simulink model "CLVF"  (R2020a)
settings: Solver=FixedStepAuto  StartTime=0.0  StopTime=tsim  FixedStep=baseRate  RelTol=1e-3  EnableMultiTasking=on
values from neighbouring files (symbols this model uses):
  a = sqrt(sum(aTimesOVec.^2))    [Run_Initializer.m]    (also in a_max_CLVF2D.m = params(4))
  a_max = 0.4/BLACKMass    [Run_Initializer.m]
  a_prime = newParams(2)    [Run_Initializer.m]    (also in a_max_LVF.m = params(2))
  acceptableRadius = 0.05    [Run_Initializer.m]
  b = newParams(3)    [Run_Initializer.m]    (also in a_max_CLVF2D.m = params(3))
  baseRate = 0.05    [Run_Initializer.m]
  BLACKMass = model_param(3)    [Run_Initializer.m]
  d = [0.16;0.542;0]    [Run_Initializer.m]    (also in a_max_LVF.m = [rotStuff(3);rotStuff(4);rotStuff(5)])
  drop_states_BLACK = rC_I0    [Run_Initializer.m]
  drop_states_BLUE = [ xLength/2+0.9; yLength/2+0.5; 0]    [Run_Initializer.m]
  drop_states_RED = rT_I0    [Run_Initializer.m]
  F_thrusters_BLACK = 0.25.*ones(8,1)    [Run_Initializer.m]
  F_thrusters_BLUE = 0.25.*ones(8,1)    [Run_Initializer.m]
  F_thrusters_RED = 0.25.*ones(8,1)    [Run_Initializer.m]
  home_states_BLACK = [ xLength/2+0.4; yLength/2; 0]    [Run_Initializer.m]
  home_states_BLUE = [ xLength/2-0.9; yLength/2+0.5; 0]    [Run_Initializer.m]
  home_states_RED = [ xLength/2-0.4; yLength/2; 0]    [Run_Initializer.m]
  init_states_BLACK = rC_I0    [Run_Initializer.m]
  init_states_BLUE = [ xLength/2+0.9; yLength/2+0.5; 0]    [Run_Initializer.m]
  init_states_RED = rT_I0    [Run_Initializer.m]
  k_v_rel = 2*v_max/a_prime    (= 1)    [Run_Initializer.m]
  ka = newParams(2)    [Run_Initializer.m]    (also in a_max_CLVF2D.m = params(2))
  kc = newParams(1)    [Run_Initializer.m]    (also in a_max_CLVF2D.m = params(1))
  kd = 5.0    (= 5)    [Run_Initializer.m]
  Kd_tb = 0.4    [Run_Initializer.m]
  Kd_tblue = 0.4    [Run_Initializer.m]
  Kd_tr = 0.4    [Run_Initializer.m]
  Kd_xb = 5    [Run_Initializer.m]
  Kd_xblue = 5    [Run_Initializer.m]
  Kd_xr = 5    [Run_Initializer.m]
  Kd_yb = 5    [Run_Initializer.m]
  Kd_yblue = 5    [Run_Initializer.m]
  Kd_yr = 5    [Run_Initializer.m]
  Kp_tb = 0.1    [Run_Initializer.m]
  Kp_tblue = 0.1    [Run_Initializer.m]
  Kp_tr = 0.1    [Run_Initializer.m]
  Kp_xb = 2    [Run_Initializer.m]
  Kp_xblue = 2    [Run_Initializer.m]
  Kp_xr = 2    [Run_Initializer.m]
  Kp_yb = 2    [Run_Initializer.m]
  Kp_yblue = 2    [Run_Initializer.m]
  Kp_yr = 2    [Run_Initializer.m]
  noise_variance_BLACK = 0    [Run_Initializer.m]
  noise_variance_BLUE = 0    [Run_Initializer.m]
  noise_variance_RED = 0    [Run_Initializer.m]
  o_hat_B = aTimesOVec./a    [Run_Initializer.m]
  o_hat_prime = o_prime/sqrt(sum(o_prime.^2))    [Run_Initializer.m]
  Phase0_End = Phase0_Duration    (= 10)    [Run_Initializer.m]
  Phase1_End = Phase0_Duration + Phase1_Duration    (= 15)    [Run_Initializer.m]
  Phase2_End = Phase0_Duration + Phase1_Duration +                                   Phase2_Duration    (= 35)    [Run_Initializer.m]
  Phase3_End = Phase0_Duration + Phase1_Duration +                                   Phase2_Duration + Phase3_Duration    [Run_Initializer.m]
  Phase3_SubPhase1_End = Phase2_End + Phase3_SubPhase1_Duration    (= 40)    [Run_Initializer.m]
  Phase3_SubPhase2_End = Phase2_End + Phase3_SubPhase1_Duration +                                   Phase3_SubPhase2_Duration    (= 45)    [Run_Initializer.m]
  Phase3_SubPhase3_End_BLACK = Phase2_End + Phase3_SubPhase1_Duration +                                   Phase3_SubPhase2_Duration +                                  Phase3_SubPhase3_Duration + Phase3_SubPhase3_and_a_half    (= 51)    [Run_Initializer.m]
  Phase3_SubPhase3_End_RED = Phase2_End + Phase3_SubPhase1_Duration +                                   Phase3_SubPhase2_Duration +                                  Phase3_SubPhase3_Duration    (= 46)    [Run_Initializer.m]
  Phase3_SubPhase4_End = Phase2_End + Phase3_SubPhase1_Duration +                                   Phase3_SubPhase2_Duration +                                  Phase3_SubPhase3_Duration +                                  Phase3_SubPhase4_Duration + Phase3_SubPhase3_and_a_half    [Run_Initializer.m]
  Phase4_End = Phase0_Duration + Phase1_Duration +                                   Phase2_Duration + Phase3_Duration +                                   Phase4_Duration    [Run_Initializer.m]
  Phase5_End = Phase0_Duration + Phase1_Duration +                                   Phase2_Duration + Phase3_Duration +                                   Phase4_Duration + Phase5_Duration    [Run_Initializer.m]
  r_co = r_co_over_a_prime*a_prime    (= 0.16)    [Run_Initializer.m]
  rC_I0 = [0.9*xLength;yLength/2-0.5;pi/2]    [Run_Initializer.m]
  rT_I0 = [yLength/2;yLength/2;possibleStarts(startingRotation)]    [Run_Initializer.m]
  serverRate = 0.1    [Run_Initializer.m]
  sys_BLACK = c2d(sys_BLACK_CONT, baseRate)    [Run_Initializer.m]
  sys_BLACK_ROT = c2d(sys_BLACK_rot_CONT, baseRate)    [Run_Initializer.m]
  sys_RED = c2d(sys_RED_CONT, baseRate)    [Run_Initializer.m]
  sys_RED_ROT = c2d(sys_RED_rot_CONT, baseRate)    [Run_Initializer.m]
  theta_d = 30*d2r    (= 0.523598775598)    [Run_Initializer.m]    (also in a_max_LVF.m = rotStuff(2))
  thruster_dist2CG_BLACK = [83.42;-52.58;55.94;-60.05;54.08;-53.92;77.06;-55.94]    [Run_Initializer.m]
  thruster_dist2CG_BLUE = [83.42;-52.58;55.94;-60.05;54.08;-53.92;77.06;-55.94]    [Run_Initializer.m]
  thruster_dist2CG_RED = [49.92;-78.08;70.46;-63.54;81.08;-50.42;57.44;-75.96]    [Run_Initializer.m]
  w_body = 6.0 * d2r    (= 0.10471975512)    [Run_Initializer.m]
undefined symbols (not defined in the file or in its folder): DiscIntNeverNeededParam, Discrete, Phase3_SubPhase3_End, platformSelection, simMode, Time, WhoAmI
libraries: dspstat3 x18, dspsigops x14, raspberrypiBasiclib x10, embdlinuxlib x8, simulink x8, ctrlSharedLib x4, mspfiltlib x3, dsparch4 x3, dspswit3 x2, MainLibrary x2, sensehatlib x1
(part 9 of 10)

== system CLVF/Grab PhaseSpace Data via UDP/Use Hardware to Obtain States/Using RED+BLACK, or RED+BLACK+ARM/Obtain BLACK States/x_dot -> x11/Hold this value ==
  In1 : Inport
  Action Port : ActionPort
  Out1 : Outport  VectorParamsAs1DForOutWhenUnconnected=off
  wires:
  In1/1 -> Out1/1

== system CLVF/Grab PhaseSpace Data via UDP/Use Hardware to Obtain States/Using RED+BLACK, or RED+BLACK+ARM/Obtain BLACK States/x_dot -> x12/Hold this value ==
  In1 : Inport
  Action Port : ActionPort
  Out1 : Outport  VectorParamsAs1DForOutWhenUnconnected=off
  wires:
  In1/1 -> Out1/1

== system CLVF/Grab PhaseSpace Data via UDP/Use Hardware to Obtain States/Using RED+BLACK, or RED+BLACK+ARM/Obtain BLACK States/x_dot -> x2/Hold this value ==
  In1 : Inport
  Action Port : ActionPort
  Out1 : Outport  VectorParamsAs1DForOutWhenUnconnected=off
  wires:
  In1/1 -> Out1/1

== system CLVF/Grab PhaseSpace Data via UDP/Use Hardware to Obtain States/Using RED+BLACK, or RED+BLACK+ARM/Obtain BLACK States/x_dot -> x3/Hold this value ==
  In1 : Inport
  Action Port : ActionPort
  Out1 : Outport  VectorParamsAs1DForOutWhenUnconnected=off
  wires:
  In1/1 -> Out1/1

== system CLVF/Grab PhaseSpace Data via UDP/Use Hardware to Obtain States/Using RED+BLACK, or RED+BLACK+ARM/Obtain BLACK States/x_dot -> x4/Hold this value ==
  In1 : Inport
  Action Port : ActionPort
  Out1 : Outport  VectorParamsAs1DForOutWhenUnconnected=off
  wires:
  In1/1 -> Out1/1

== system CLVF/Grab PhaseSpace Data via UDP/Use Hardware to Obtain States/Using RED+BLACK, or RED+BLACK+ARM/Obtain BLACK States/x_dot -> x5/Hold this value ==
  In1 : Inport
  Action Port : ActionPort
  Out1 : Outport  VectorParamsAs1DForOutWhenUnconnected=off
  wires:
  In1/1 -> Out1/1

== system CLVF/Grab PhaseSpace Data via UDP/Use Hardware to Obtain States/Using RED+BLACK, or RED+BLACK+ARM/Obtain BLACK States/x_dot -> x6/Hold this value ==
  In1 : Inport
  Action Port : ActionPort
  Out1 : Outport  VectorParamsAs1DForOutWhenUnconnected=off
  wires:
  In1/1 -> Out1/1

== system CLVF/Grab PhaseSpace Data via UDP/Use Hardware to Obtain States/Using RED+BLACK, or RED+BLACK+ARM/Obtain BLACK States/x_dot -> x7/Hold this value ==
  In1 : Inport
  Action Port : ActionPort
  Out1 : Outport  VectorParamsAs1DForOutWhenUnconnected=off
  wires:
  In1/1 -> Out1/1

== system CLVF/Grab PhaseSpace Data via UDP/Use Hardware to Obtain States/Using RED+BLACK, or RED+BLACK+ARM/Obtain BLACK States/x_dot -> x8/Hold this value ==
  In1 : Inport
  Action Port : ActionPort
  Out1 : Outport  VectorParamsAs1DForOutWhenUnconnected=off
  wires:
  In1/1 -> Out1/1

== system CLVF/Grab PhaseSpace Data via UDP/Use Hardware to Obtain States/Using RED+BLACK, or RED+BLACK+ARM/Obtain BLACK States/x_dot -> x9/Hold this value ==
  In1 : Inport
  Action Port : ActionPort
  Out1 : Outport  VectorParamsAs1DForOutWhenUnconnected=off
  wires:
  In1/1 -> Out1/1

== system CLVF/Grab PhaseSpace Data via UDP/Use Hardware to Obtain States/Using RED+BLACK, or RED+BLACK+ARM/Obtain RED States/Correct Time/Enabled Subsystem ==
  In1 : Inport
  Enable : EnablePort
  Out1 : Outport  VectorParamsAs1DForOutWhenUnconnected=off
  wires:
  In1/1 -> Out1/1

== system CLVF/Grab PhaseSpace Data via UDP/Use Hardware to Obtain States/Using RED+BLACK, or RED+BLACK+ARM/Obtain RED States/x_dot -> x1/Hold this value ==
  In1 : Inport
  Action Port : ActionPort
  Out1 : Outport  VectorParamsAs1DForOutWhenUnconnected=off
  wires:
  In1/1 -> Out1/1

== system CLVF/Grab PhaseSpace Data via UDP/Use Hardware to Obtain States/Using RED+BLACK, or RED+BLACK+ARM/Obtain RED States/x_dot -> x10/Hold this value ==
  In1 : Inport
  Action Port : ActionPort
  Out1 : Outport  VectorParamsAs1DForOutWhenUnconnected=off
  wires:
  In1/1 -> Out1/1

== system CLVF/Grab PhaseSpace Data via UDP/Use Hardware to Obtain States/Using RED+BLACK, or RED+BLACK+ARM/Obtain RED States/x_dot -> x11/Hold this value ==
  In1 : Inport
  Action Port : ActionPort
  Out1 : Outport  VectorParamsAs1DForOutWhenUnconnected=off
  wires:
  In1/1 -> Out1/1

== system CLVF/Grab PhaseSpace Data via UDP/Use Hardware to Obtain States/Using RED+BLACK, or RED+BLACK+ARM/Obtain RED States/x_dot -> x12/Hold this value ==
  In1 : Inport
  Action Port : ActionPort
  Out1 : Outport  VectorParamsAs1DForOutWhenUnconnected=off
  wires:
  In1/1 -> Out1/1

== system CLVF/Grab PhaseSpace Data via UDP/Use Hardware to Obtain States/Using RED+BLACK, or RED+BLACK+ARM/Obtain RED States/x_dot -> x2/Hold this value ==
  In1 : Inport
  Action Port : ActionPort
  Out1 : Outport  VectorParamsAs1DForOutWhenUnconnected=off
  wires:
  In1/1 -> Out1/1

== system CLVF/Grab PhaseSpace Data via UDP/Use Hardware to Obtain States/Using RED+BLACK, or RED+BLACK+ARM/Obtain RED States/x_dot -> x3/Hold this value ==
  In1 : Inport
  Action Port : ActionPort
  Out1 : Outport  VectorParamsAs1DForOutWhenUnconnected=off
  wires:
  In1/1 -> Out1/1

== system CLVF/Grab PhaseSpace Data via UDP/Use Hardware to Obtain States/Using RED+BLACK, or RED+BLACK+ARM/Obtain RED States/x_dot -> x4/Hold this value ==
  In1 : Inport
  Action Port : ActionPort
  Out1 : Outport  VectorParamsAs1DForOutWhenUnconnected=off
  wires:
  In1/1 -> Out1/1

== system CLVF/Grab PhaseSpace Data via UDP/Use Hardware to Obtain States/Using RED+BLACK, or RED+BLACK+ARM/Obtain RED States/x_dot -> x5/Hold this value ==
  In1 : Inport
  Action Port : ActionPort
  Out1 : Outport  VectorParamsAs1DForOutWhenUnconnected=off
  wires:
  In1/1 -> Out1/1

== system CLVF/Grab PhaseSpace Data via UDP/Use Hardware to Obtain States/Using RED+BLACK, or RED+BLACK+ARM/Obtain RED States/x_dot -> x6/Hold this value ==
  In1 : Inport
  Action Port : ActionPort
  Out1 : Outport  VectorParamsAs1DForOutWhenUnconnected=off
  wires:
  In1/1 -> Out1/1

== system CLVF/Grab PhaseSpace Data via UDP/Use Hardware to Obtain States/Using RED+BLACK, or RED+BLACK+ARM/Obtain RED States/x_dot -> x7/Hold this value ==
  In1 : Inport
  Action Port : ActionPort
  Out1 : Outport  VectorParamsAs1DForOutWhenUnconnected=off
  wires:
  In1/1 -> Out1/1

== system CLVF/Grab PhaseSpace Data via UDP/Use Hardware to Obtain States/Using RED+BLACK, or RED+BLACK+ARM/Obtain RED States/x_dot -> x8/Hold this value ==
  In1 : Inport
  Action Port : ActionPort
  Out1 : Outport  VectorParamsAs1DForOutWhenUnconnected=off
  wires:
  In1/1 -> Out1/1

== system CLVF/Grab PhaseSpace Data via UDP/Use Hardware to Obtain States/Using RED+BLACK, or RED+BLACK+ARM/Obtain RED States/x_dot -> x9/Hold this value ==
  In1 : Inport
  Action Port : ActionPort
  Out1 : Outport  VectorParamsAs1DForOutWhenUnconnected=off
  wires:
  In1/1 -> Out1/1

== system CLVF/Phase #3: Experiment/Change BLACK Behavior/Sub-Phase #1/Custom Discrete PD (Attitude)/x_dot -> x1/Hold this value ==
  In1 : Inport
  Action Port : ActionPort  ActionPortLabel=if(u1 ~= 0)
  Out1 : Outport  VectorParamsAs1DForOutWhenUnconnected=off
  wires:
  In1/1 -> Out1/1

== system CLVF/Phase #3: Experiment/Change BLACK Behavior/Sub-Phase #1/Custom Discrete PD (X-Position)/x_dot -> x1/Hold this value ==
  In1 : Inport
  Action Port : ActionPort  ActionPortLabel=if(u1 ~= 0)
  Out1 : Outport  VectorParamsAs1DForOutWhenUnconnected=off
  wires:
  In1/1 -> Out1/1

== system CLVF/Phase #3: Experiment/Change BLACK Behavior/Sub-Phase #1/Custom Discrete PD (Y-Position)/x_dot -> x1/Hold this value ==
  In1 : Inport
  Action Port : ActionPort  ActionPortLabel=if(u1 ~= 0)
  Out1 : Outport  VectorParamsAs1DForOutWhenUnconnected=off
  wires:
  In1/1 -> Out1/1

== system CLVF/Phase #3: Experiment/Change BLACK Behavior/Sub-Phase #4/Custom Discrete PD (Attitude)/x_dot -> x1/Hold this value ==
  In1 : Inport
  Action Port : ActionPort  ActionPortLabel=if(u1 ~= 0)
  Out1 : Outport  VectorParamsAs1DForOutWhenUnconnected=off
  wires:
  In1/1 -> Out1/1

== system CLVF/Phase #3: Experiment/Change BLACK Behavior/Sub-Phase #4/Lyapunov GNC/CLVF Approach/Vec Derivative ==
  In1 : Inport
  Demux4 : Demux  Outputs=3
  Mux : Mux  Inputs=3
  "x_dot -> x1" : Subsystem
  "x_dot -> x2" : Subsystem
  "x_dot -> x3" : Subsystem
  Out1 : Outport  VectorParamsAs1DForOutWhenUnconnected=off
  wires:
  Demux4/1 -> "x_dot -> x1"/1(y(t))
  Demux4/2 -> "x_dot -> x2"/1(y(t))
  Demux4/3 -> "x_dot -> x3"/1(y(t))
  "x_dot -> x2"/1(dy(t)/dt) -> Mux/2
  In1/1 -> Demux4/1
  Mux/1 -> Out1/1
  "x_dot -> x1"/1(dy(t)/dt) -> Mux/1
  "x_dot -> x3"/1(dy(t)/dt) -> Mux/3

== system CLVF/Phase #3: Experiment/Change BLACK Behavior/Sub-Phase #4/Lyapunov GNC/Lyapunov/Vec Derivative ==
  In1 : Inport
  Demux4 : Demux  Outputs=3
  Mux : Mux  Inputs=3
  "x_dot -> x1" : Subsystem
  "x_dot -> x2" : Subsystem
  "x_dot -> x3" : Subsystem
  Out1 : Outport  VectorParamsAs1DForOutWhenUnconnected=off
  wires:
  Demux4/1 -> "x_dot -> x1"/1(y(t))
  Demux4/2 -> "x_dot -> x2"/1(y(t))
  Demux4/3 -> "x_dot -> x3"/1(y(t))
  "x_dot -> x2"/1(dy(t)/dt) -> Mux/2
  In1/1 -> Demux4/1
  Mux/1 -> Out1/1
  "x_dot -> x1"/1(dy(t)/dt) -> Mux/1
  "x_dot -> x3"/1(dy(t)/dt) -> Mux/3

== system CLVF/Phase #3: Experiment/Change BLACK Behavior/Sub-Phase #4/Lyapunov GNC/Navigation/Vec Derivative ==
  In1 : Inport
  Demux4 : Demux  Outputs=3
  Mux : Mux  Inputs=3
  "x_dot -> x1" : Subsystem
  "x_dot -> x2" : Subsystem
  "x_dot -> x3" : Subsystem
  Out1 : Outport  VectorParamsAs1DForOutWhenUnconnected=off
  wires:
  Demux4/1 -> "x_dot -> x1"/1(y(t))
  Demux4/2 -> "x_dot -> x2"/1(y(t))
  Demux4/3 -> "x_dot -> x3"/1(y(t))
  "x_dot -> x2"/1(dy(t)/dt) -> Mux/2
  In1/1 -> Demux4/1
  Mux/1 -> Out1/1
  "x_dot -> x1"/1(dy(t)/dt) -> Mux/1
  "x_dot -> x3"/1(dy(t)/dt) -> Mux/3

== system CLVF/Phase #3: Experiment/Change BLACK Behavior/Sub-Phase #4/Lyapunov GNC/Navigation/Vec Derivative1 ==
  In1 : Inport
  Demux4 : Demux  Outputs=3
  Mux : Mux  Inputs=3
  "x_dot -> x1" : Subsystem
  "x_dot -> x2" : Subsystem
  "x_dot -> x3" : Subsystem
  Out1 : Outport  VectorParamsAs1DForOutWhenUnconnected=off
  wires:
  Demux4/1 -> "x_dot -> x1"/1(y(t))
  Demux4/2 -> "x_dot -> x2"/1(y(t))
  Demux4/3 -> "x_dot -> x3"/1(y(t))
  "x_dot -> x2"/1(dy(t)/dt) -> Mux/2
  In1/1 -> Demux4/1
  Mux/1 -> Out1/1
  "x_dot -> x1"/1(dy(t)/dt) -> Mux/1
  "x_dot -> x3"/1(dy(t)/dt) -> Mux/3

== system CLVF/Phase #3: Experiment/Change BLACK Behavior/Sub-Phase #4/Lyapunov GNC/Navigation/tau_km1_BLACK ==
  Constant : Constant  Value=serverRate
  Data Store Read : DataStoreRead  DataStoreName=BLACK_Tz_Sat
  Data Store Read2 : DataStoreRead  DataStoreName=Univ_Time
  Delay : Delay  DelayLength=1  SampleTime=baseRate
  MATLAB Function : MATLAB Function  TreatAsAtomicUnit=on
  Sample and Hold : dspsigops/Sample and Hold  trig=Rising edge  initCond=0  latchinput=off
  ukm1 : Outport  VectorParamsAs1DForOutWhenUnconnected=off
  wires:
  Sample and Hold/1 -> ukm1/1
  Data Store Read2/1 -> MATLAB Function/1(TIME)
  MATLAB Function/1(y) -> Sample and Hold/Trigger
  Constant/1 -> MATLAB Function/2(SERVER)
  Data Store Read/1 -> Delay/1
  Delay/1 -> Sample and Hold/1

== system CLVF/Phase #3: Experiment/Change BLACK Behavior/Sub-Phase #4/Lyapunov GNC/Navigation/tau_km1_RED ==
  Constant : Constant  Value=serverRate
  Data Store Read : DataStoreRead  DataStoreName=RED_Tz_Sat
  Data Store Read2 : DataStoreRead  DataStoreName=Univ_Time
  Delay1 : Delay  DelayLength=1  SampleTime=baseRate
  MATLAB Function : MATLAB Function  TreatAsAtomicUnit=on
  Sample and Hold : dspsigops/Sample and Hold  trig=Rising edge  initCond=0  latchinput=off
  ukm1 : Outport  VectorParamsAs1DForOutWhenUnconnected=off
  wires:
  Sample and Hold/1 -> ukm1/1
  Data Store Read2/1 -> MATLAB Function/1(TIME)
  MATLAB Function/1(y) -> Sample and Hold/Trigger
  Constant/1 -> MATLAB Function/2(SERVER)
  Data Store Read/1 -> Delay1/1
  Delay1/1 -> Sample and Hold/1

== system CLVF/Phase #3: Experiment/Change BLACK Behavior/Sub-Phase #4/Lyapunov GNC/Navigation/u_km1_BLACK ==
  Constant : Constant  Value=serverRate
  Constant1 : Constant  Value=0
  Data Store Read : DataStoreRead  DataStoreName=BLACK_Fx_Sat
  Data Store Read1 : DataStoreRead  DataStoreName=BLACK_Fy_Sat
  Data Store Read2 : DataStoreRead  DataStoreName=Univ_Time
  Delay : Delay  DelayLength=1  SampleTime=baseRate
  Delay1 : Delay  DelayLength=1  SampleTime=baseRate
  MATLAB Function : MATLAB Function  TreatAsAtomicUnit=on
  Mux : Mux  Inputs=3
  Sample and Hold : dspsigops/Sample and Hold  trig=Rising edge  initCond=0  latchinput=off
  ukm1 : Outport  VectorParamsAs1DForOutWhenUnconnected=off
  wires:
  Data Store Read1/1 -> Delay1/1
  Data Store Read/1 -> Delay/1
  Constant1/1 -> Mux/3
  Mux/1 -> Sample and Hold/1
  Sample and Hold/1 -> ukm1/1
  Data Store Read2/1 -> MATLAB Function/1(TIME)
  MATLAB Function/1(y) -> Sample and Hold/Trigger
  Constant/1 -> MATLAB Function/2(SERVER)
  Delay/1 -> Mux/1
  Delay1/1 -> Mux/2

== system CLVF/Phase #3: Experiment/Change BLACK Behavior/Sub-Phase #4/Lyapunov GNC/Navigation/u_km1_RED ==
  Constant : Constant  Value=serverRate
  Constant1 : Constant  Value=0
  Data Store Read : DataStoreRead  DataStoreName=RED_Fx_Sat
  Data Store Read1 : DataStoreRead  DataStoreName=RED_Fy_Sat
  Data Store Read2 : DataStoreRead  DataStoreName=Univ_Time
  Delay : Delay  DelayLength=1  SampleTime=baseRate
  Delay1 : Delay  DelayLength=1  SampleTime=baseRate
  MATLAB Function : MATLAB Function  TreatAsAtomicUnit=on
  Mux : Mux  Inputs=3
  Sample and Hold : dspsigops/Sample and Hold  trig=Rising edge  initCond=0  latchinput=off
  ukm1 : Outport  VectorParamsAs1DForOutWhenUnconnected=off
  wires:
  Data Store Read/1 -> Delay/1
  Delay1/1 -> Mux/2
  Data Store Read1/1 -> Delay1/1
  Delay/1 -> Mux/1
  Constant1/1 -> Mux/3
  Mux/1 -> Sample and Hold/1
  Sample and Hold/1 -> ukm1/1
  Data Store Read2/1 -> MATLAB Function/1(TIME)
  MATLAB Function/1(y) -> Sample and Hold/Trigger
  Constant/1 -> MATLAB Function/2(SERVER)

== system CLVF/Phase #3: Experiment/Change BLACK Behavior/Sub-Phase #4/Lyapunov GNC/Navigation/x_dot -> x1 ==
  note: dy/dt ~= (y2-y1)/deltaT
  y(t) : Inport
  Delay1 : Delay  DelayLength=1  InitialConditionSource=Input port
      settings: InputPortMap=u0,p4
  Hold this value : Subsystem  TreatAsAtomicUnit=on
  Sum6 : Sum  Inputs=-+|
  divide by delta T : Gain  Gain=1/serverRate
  "if we went through a \"step\"" : If  IfExpression=u1 ~= 0  ShowElse=off
  dy(t)/dt : Outport  VectorParamsAs1DForOutWhenUnconnected=off
  wires:
  divide by delta T/1 -> dy(t)/dt/1
  Delay1/1 -> Sum6/1
  "if we went through a \"step\""/1 -> Hold this value/Action
  Hold this value/1(Out1) -> divide by delta T/1
  Sum6/1 -> "if we went through a \"step\""/1, Hold this value/1(In1)
  y(t)/1 -> Sum6/2, Delay1/2, Delay1/1

== system CLVF/Phase #3: Experiment/Change BLACK Behavior/Sub-Phase #4/Lyapunov GNC/Navigation/x_dot -> x3 ==
  note: dy/dt ~= (y2-y1)/deltaT
  y(t) : Inport
  Delay1 : Delay  DelayLength=1  InitialConditionSource=Input port
      settings: InputPortMap=u0,p4
  Hold this value : Subsystem  TreatAsAtomicUnit=on
  Sum6 : Sum  Inputs=-+|
  divide by delta T : Gain  Gain=1/serverRate
  "if we went through a \"step\"" : If  IfExpression=u1 ~= 0  ShowElse=off
  dy(t)/dt : Outport  VectorParamsAs1DForOutWhenUnconnected=off
  wires:
  divide by delta T/1 -> dy(t)/dt/1
  Delay1/1 -> Sum6/1
  "if we went through a \"step\""/1 -> Hold this value/Action
  Hold this value/1(Out1) -> divide by delta T/1
  Sum6/1 -> "if we went through a \"step\""/1, Hold this value/1(In1)
  y(t)/1 -> Sum6/2, Delay1/2, Delay1/1

== system CLVF/Phase #3: Experiment/Change BLUE Behavior/Sub-Phase #1/Custom Discrete PD (Attitude)/x_dot -> x1/Hold this value ==
  In1 : Inport
  Action Port : ActionPort  ActionPortLabel=if(u1 ~= 0)
  Out1 : Outport  VectorParamsAs1DForOutWhenUnconnected=off
  wires:
  In1/1 -> Out1/1

== system CLVF/Phase #3: Experiment/Change BLUE Behavior/Sub-Phase #1/Custom Discrete PD (X-Position)/x_dot -> x1/Hold this value ==
  In1 : Inport
  Action Port : ActionPort  ActionPortLabel=if(u1 ~= 0)
  Out1 : Outport  VectorParamsAs1DForOutWhenUnconnected=off
  wires:
  In1/1 -> Out1/1

== system CLVF/Phase #3: Experiment/Change BLUE Behavior/Sub-Phase #1/Custom Discrete PD (Y-Position)/x_dot -> x1/Hold this value ==
  In1 : Inport
  Action Port : ActionPort  ActionPortLabel=if(u1 ~= 0)
  Out1 : Outport  VectorParamsAs1DForOutWhenUnconnected=off
  wires:
  In1/1 -> Out1/1

== system CLVF/Phase #3: Experiment/Change BLUE Behavior/Sub-Phase #4/Custom Discrete PD (Attitude)/x_dot -> x1/Hold this value ==
  In1 : Inport
  Action Port : ActionPort  ActionPortLabel=if(u1 ~= 0)
  Out1 : Outport  VectorParamsAs1DForOutWhenUnconnected=off
  wires:
  In1/1 -> Out1/1

== system CLVF/Phase #3: Experiment/Change BLUE Behavior/Sub-Phase #4/Custom Discrete PD (X-Position)/x_dot -> x1/Hold this value ==
  In1 : Inport
  Action Port : ActionPort  ActionPortLabel=if(u1 ~= 0)
  Out1 : Outport  VectorParamsAs1DForOutWhenUnconnected=off
  wires:
  In1/1 -> Out1/1

== system CLVF/Phase #3: Experiment/Change BLUE Behavior/Sub-Phase #4/Custom Discrete PD (Y-Position)/x_dot -> x1/Hold this value ==
  In1 : Inport
  Action Port : ActionPort  ActionPortLabel=if(u1 ~= 0)
  Out1 : Outport  VectorParamsAs1DForOutWhenUnconnected=off
  wires:
  In1/1 -> Out1/1

== system CLVF/Phase #3: Experiment/Change RED Behavior/Sub-Phase #1/Custom Discrete PD (Attitude)/x_dot -> x1/Hold this value ==
  In1 : Inport
  Action Port : ActionPort  ActionPortLabel=if(u1 ~= 0)
  Out1 : Outport  VectorParamsAs1DForOutWhenUnconnected=off
  wires:
  In1/1 -> Out1/1

== system CLVF/Phase #3: Experiment/Change RED Behavior/Sub-Phase #1/Custom Discrete PD (X-Position)/x_dot -> x1/Hold this value ==
  In1 : Inport
  Action Port : ActionPort  ActionPortLabel=if(u1 ~= 0)
  Out1 : Outport  VectorParamsAs1DForOutWhenUnconnected=off
  wires:
  In1/1 -> Out1/1

== system CLVF/Phase #3: Experiment/Change RED Behavior/Sub-Phase #1/Custom Discrete PD (Y-Position)/x_dot -> x1/Hold this value ==
  In1 : Inport
  Action Port : ActionPort  ActionPortLabel=if(u1 ~= 0)
  Out1 : Outport  VectorParamsAs1DForOutWhenUnconnected=off
  wires:
  In1/1 -> Out1/1

== system CLVF/Phase #3: Experiment/Change RED Behavior/Sub-Phase #4/Custom Discrete PD (Attitude)/x_dot -> x1/Hold this value ==
  In1 : Inport
  Action Port : ActionPort  ActionPortLabel=if(u1 ~= 0)
  Out1 : Outport  VectorParamsAs1DForOutWhenUnconnected=off
  wires:
  In1/1 -> Out1/1

== system CLVF/Phase #3: Experiment/Change RED Behavior/Sub-Phase #4/Custom Discrete PD (X-Position)/x_dot -> x1/Hold this value ==
  In1 : Inport
  Action Port : ActionPort  ActionPortLabel=if(u1 ~= 0)
  Out1 : Outport  VectorParamsAs1DForOutWhenUnconnected=off
  wires:
  In1/1 -> Out1/1

== system CLVF/Phase #3: Experiment/Change RED Behavior/Sub-Phase #4/Custom Discrete PD (Y-Position)/x_dot -> x1/Hold this value ==
  In1 : Inport
  Action Port : ActionPort  ActionPortLabel=if(u1 ~= 0)
  Out1 : Outport  VectorParamsAs1DForOutWhenUnconnected=off
  wires:
  In1/1 -> Out1/1

== system CLVF/Phase #3: Experiment/Change BLACK Behavior/Sub-Phase #4/Lyapunov GNC/CLVF Approach/Vec Derivative/x_dot -> x1 ==
  note: dy/dt ~= (y2-y1)/deltaT
  y(t) : Inport
  Delay1 : Delay  DelayLength=1  InitialConditionSource=Input port
      settings: InputPortMap=u0,p4
  Hold this value : Subsystem  TreatAsAtomicUnit=on
  Sum6 : Sum  Inputs=-+|
  divide by delta T : Gain  Gain=1/serverRate
  "if we went through a \"step\"" : If  IfExpression=u1 ~= 0  ShowElse=off
  dy(t)/dt : Outport  VectorParamsAs1DForOutWhenUnconnected=off
  wires:
  divide by delta T/1 -> dy(t)/dt/1
  Delay1/1 -> Sum6/1
  "if we went through a \"step\""/1 -> Hold this value/Action
  Hold this value/1(Out1) -> divide by delta T/1
  Sum6/1 -> "if we went through a \"step\""/1, Hold this value/1(In1)
  y(t)/1 -> Sum6/2, Delay1/2, Delay1/1

== system CLVF/Phase #3: Experiment/Change BLACK Behavior/Sub-Phase #4/Lyapunov GNC/CLVF Approach/Vec Derivative/x_dot -> x2 ==
  note: dy/dt ~= (y2-y1)/deltaT
  y(t) : Inport
  Delay1 : Delay  DelayLength=1  InitialConditionSource=Input port
      settings: InputPortMap=u0,p4
  Hold this value : Subsystem  TreatAsAtomicUnit=on
  Sum6 : Sum  Inputs=-+|
  divide by delta T : Gain  Gain=1/serverRate
  "if we went through a \"step\"" : If  IfExpression=u1 ~= 0  ShowElse=off
  dy(t)/dt : Outport  VectorParamsAs1DForOutWhenUnconnected=off
  wires:
  divide by delta T/1 -> dy(t)/dt/1
  Delay1/1 -> Sum6/1
  "if we went through a \"step\""/1 -> Hold this value/Action
  Hold this value/1(Out1) -> divide by delta T/1
  Sum6/1 -> "if we went through a \"step\""/1, Hold this value/1(In1)
  y(t)/1 -> Sum6/2, Delay1/2, Delay1/1

== system CLVF/Phase #3: Experiment/Change BLACK Behavior/Sub-Phase #4/Lyapunov GNC/CLVF Approach/Vec Derivative/x_dot -> x3 ==
  note: dy/dt ~= (y2-y1)/deltaT
  y(t) : Inport
  Delay1 : Delay  DelayLength=1  InitialConditionSource=Input port
      settings: InputPortMap=u0,p4
  Hold this value : Subsystem  TreatAsAtomicUnit=on
  Sum6 : Sum  Inputs=-+|
  divide by delta T : Gain  Gain=1/serverRate
  "if we went through a \"step\"" : If  IfExpression=u1 ~= 0  ShowElse=off
  dy(t)/dt : Outport  VectorParamsAs1DForOutWhenUnconnected=off
  wires:
  divide by delta T/1 -> dy(t)/dt/1
  Delay1/1 -> Sum6/1
  "if we went through a \"step\""/1 -> Hold this value/Action
  Hold this value/1(Out1) -> divide by delta T/1
  Sum6/1 -> "if we went through a \"step\""/1, Hold this value/1(In1)
  y(t)/1 -> Sum6/2, Delay1/2, Delay1/1

== system CLVF/Phase #3: Experiment/Change BLACK Behavior/Sub-Phase #4/Lyapunov GNC/Lyapunov/Vec Derivative/x_dot -> x1 ==
  note: dy/dt ~= (y2-y1)/deltaT
  y(t) : Inport
  Delay1 : Delay  DelayLength=1  InitialConditionSource=Input port
      settings: InputPortMap=u0,p4
  Hold this value : Subsystem  TreatAsAtomicUnit=on
  Sum6 : Sum  Inputs=-+|
  divide by delta T : Gain  Gain=1/serverRate
  "if we went through a \"step\"" : If  IfExpression=u1 ~= 0  ShowElse=off
  dy(t)/dt : Outport  VectorParamsAs1DForOutWhenUnconnected=off
  wires:
  divide by delta T/1 -> dy(t)/dt/1
  Delay1/1 -> Sum6/1
  "if we went through a \"step\""/1 -> Hold this value/Action
  Hold this value/1(Out1) -> divide by delta T/1
  Sum6/1 -> "if we went through a \"step\""/1, Hold this value/1(In1)
  y(t)/1 -> Sum6/2, Delay1/2, Delay1/1

== system CLVF/Phase #3: Experiment/Change BLACK Behavior/Sub-Phase #4/Lyapunov GNC/Lyapunov/Vec Derivative/x_dot -> x2 ==
  note: dy/dt ~= (y2-y1)/deltaT
  y(t) : Inport
  Delay1 : Delay  DelayLength=1  InitialConditionSource=Input port
      settings: InputPortMap=u0,p4
  Hold this value : Subsystem  TreatAsAtomicUnit=on
  Sum6 : Sum  Inputs=-+|
  divide by delta T : Gain  Gain=1/serverRate
  "if we went through a \"step\"" : If  IfExpression=u1 ~= 0  ShowElse=off
  dy(t)/dt : Outport  VectorParamsAs1DForOutWhenUnconnected=off
  wires:
  divide by delta T/1 -> dy(t)/dt/1
  Delay1/1 -> Sum6/1
  "if we went through a \"step\""/1 -> Hold this value/Action
  Hold this value/1(Out1) -> divide by delta T/1
  Sum6/1 -> "if we went through a \"step\""/1, Hold this value/1(In1)
  y(t)/1 -> Delay1/2, Delay1/1, Sum6/2

== system CLVF/Phase #3: Experiment/Change BLACK Behavior/Sub-Phase #4/Lyapunov GNC/Lyapunov/Vec Derivative/x_dot -> x3 ==
  note: dy/dt ~= (y2-y1)/deltaT
  y(t) : Inport
  Delay1 : Delay  DelayLength=1  InitialConditionSource=Input port
      settings: InputPortMap=u0,p4
  Hold this value : Subsystem  TreatAsAtomicUnit=on
  Sum6 : Sum  Inputs=-+|
  divide by delta T : Gain  Gain=1/serverRate
  "if we went through a \"step\"" : If  IfExpression=u1 ~= 0  ShowElse=off
  dy(t)/dt : Outport  VectorParamsAs1DForOutWhenUnconnected=off
  wires:
  divide by delta T/1 -> dy(t)/dt/1
  Delay1/1 -> Sum6/1
  "if we went through a \"step\""/1 -> Hold this value/Action
  Hold this value/1(Out1) -> divide by delta T/1
  Sum6/1 -> "if we went through a \"step\""/1, Hold this value/1(In1)
  y(t)/1 -> Sum6/2, Delay1/2, Delay1/1

== system CLVF/Phase #3: Experiment/Change BLACK Behavior/Sub-Phase #4/Lyapunov GNC/Navigation/Vec Derivative/x_dot -> x1 ==
  note: dy/dt ~= (y2-y1)/deltaT
  y(t) : Inport
  Delay1 : Delay  DelayLength=1  InitialConditionSource=Input port
      settings: InputPortMap=u0,p4
  Hold this value : Subsystem  TreatAsAtomicUnit=on
  Sum6 : Sum  Inputs=-+|
  divide by delta T : Gain  Gain=1/serverRate
  "if we went through a \"step\"" : If  IfExpression=u1 ~= 0  ShowElse=off
  dy(t)/dt : Outport  VectorParamsAs1DForOutWhenUnconnected=off
  wires:
  divide by delta T/1 -> dy(t)/dt/1
  Delay1/1 -> Sum6/1
  "if we went through a \"step\""/1 -> Hold this value/Action
  Hold this value/1(Out1) -> divide by delta T/1
  Sum6/1 -> "if we went through a \"step\""/1, Hold this value/1(In1)
  y(t)/1 -> Sum6/2, Delay1/2, Delay1/1

== system CLVF/Phase #3: Experiment/Change BLACK Behavior/Sub-Phase #4/Lyapunov GNC/Navigation/Vec Derivative/x_dot -> x2 ==
  note: dy/dt ~= (y2-y1)/deltaT
  y(t) : Inport
  Delay1 : Delay  DelayLength=1  InitialConditionSource=Input port
      settings: InputPortMap=u0,p4
  Hold this value : Subsystem  TreatAsAtomicUnit=on
  Sum6 : Sum  Inputs=-+|
  divide by delta T : Gain  Gain=1/serverRate
  "if we went through a \"step\"" : If  IfExpression=u1 ~= 0  ShowElse=off
  dy(t)/dt : Outport  VectorParamsAs1DForOutWhenUnconnected=off
  wires:
  divide by delta T/1 -> dy(t)/dt/1
  Delay1/1 -> Sum6/1
  "if we went through a \"step\""/1 -> Hold this value/Action
  Hold this value/1(Out1) -> divide by delta T/1
  Sum6/1 -> "if we went through a \"step\""/1, Hold this value/1(In1)
  y(t)/1 -> Sum6/2, Delay1/2, Delay1/1

== system CLVF/Phase #3: Experiment/Change BLACK Behavior/Sub-Phase #4/Lyapunov GNC/Navigation/Vec Derivative/x_dot -> x3 ==
  note: dy/dt ~= (y2-y1)/deltaT
  y(t) : Inport
  Delay1 : Delay  DelayLength=1  InitialConditionSource=Input port
      settings: InputPortMap=u0,p4
  Hold this value : Subsystem  TreatAsAtomicUnit=on
  Sum6 : Sum  Inputs=-+|
  divide by delta T : Gain  Gain=1/serverRate
  "if we went through a \"step\"" : If  IfExpression=u1 ~= 0  ShowElse=off
  dy(t)/dt : Outport  VectorParamsAs1DForOutWhenUnconnected=off
  wires:
  divide by delta T/1 -> dy(t)/dt/1
  Delay1/1 -> Sum6/1
  "if we went through a \"step\""/1 -> Hold this value/Action
  Hold this value/1(Out1) -> divide by delta T/1
  Sum6/1 -> "if we went through a \"step\""/1, Hold this value/1(In1)
  y(t)/1 -> Sum6/2, Delay1/2, Delay1/1

== system CLVF/Phase #3: Experiment/Change BLACK Behavior/Sub-Phase #4/Lyapunov GNC/Navigation/Vec Derivative1/x_dot -> x1 ==
  note: dy/dt ~= (y2-y1)/deltaT
  y(t) : Inport
  Delay1 : Delay  DelayLength=1  InitialConditionSource=Input port
      settings: InputPortMap=u0,p4
  Hold this value : Subsystem  TreatAsAtomicUnit=on
  Sum6 : Sum  Inputs=-+|
  divide by delta T : Gain  Gain=1/serverRate
  "if we went through a \"step\"" : If  IfExpression=u1 ~= 0  ShowElse=off
  dy(t)/dt : Outport  VectorParamsAs1DForOutWhenUnconnected=off
  wires:
  divide by delta T/1 -> dy(t)/dt/1
  Delay1/1 -> Sum6/1
  "if we went through a \"step\""/1 -> Hold this value/Action
  Hold this value/1(Out1) -> divide by delta T/1
  Sum6/1 -> "if we went through a \"step\""/1, Hold this value/1(In1)
  y(t)/1 -> Sum6/2, Delay1/2, Delay1/1

== system CLVF/Phase #3: Experiment/Change BLACK Behavior/Sub-Phase #4/Lyapunov GNC/Navigation/Vec Derivative1/x_dot -> x2 ==
  note: dy/dt ~= (y2-y1)/deltaT
  y(t) : Inport
  Delay1 : Delay  DelayLength=1  InitialConditionSource=Input port
      settings: InputPortMap=u0,p4
  Hold this value : Subsystem  TreatAsAtomicUnit=on
  Sum6 : Sum  Inputs=-+|
  divide by delta T : Gain  Gain=1/serverRate
  "if we went through a \"step\"" : If  IfExpression=u1 ~= 0  ShowElse=off
  dy(t)/dt : Outport  VectorParamsAs1DForOutWhenUnconnected=off
  wires:
  divide by delta T/1 -> dy(t)/dt/1
  Delay1/1 -> Sum6/1
  "if we went through a \"step\""/1 -> Hold this value/Action
  Hold this value/1(Out1) -> divide by delta T/1
  Sum6/1 -> "if we went through a \"step\""/1, Hold this value/1(In1)
  y(t)/1 -> Sum6/2, Delay1/2, Delay1/1

== system CLVF/Phase #3: Experiment/Change BLACK Behavior/Sub-Phase #4/Lyapunov GNC/Navigation/Vec Derivative1/x_dot -> x3 ==
  note: dy/dt ~= (y2-y1)/deltaT
  y(t) : Inport
  Delay1 : Delay  DelayLength=1  InitialConditionSource=Input port
      settings: InputPortMap=u0,p4
  Hold this value : Subsystem  TreatAsAtomicUnit=on
  Sum6 : Sum  Inputs=-+|
  divide by delta T : Gain  Gain=1/serverRate
  "if we went through a \"step\"" : If  IfExpression=u1 ~= 0  ShowElse=off
  dy(t)/dt : Outport  VectorParamsAs1DForOutWhenUnconnected=off
  wires:
  divide by delta T/1 -> dy(t)/dt/1
  Delay1/1 -> Sum6/1
  "if we went through a \"step\""/1 -> Hold this value/Action
  Hold this value/1(Out1) -> divide by delta T/1
  Sum6/1 -> "if we went through a \"step\""/1, Hold this value/1(In1)
  y(t)/1 -> Sum6/2, Delay1/2, Delay1/1

== system CLVF/Phase #3: Experiment/Change BLACK Behavior/Sub-Phase #4/Lyapunov GNC/Navigation/x_dot -> x1/Hold this value ==
  In1 : Inport
  Action Port : ActionPort  ActionPortLabel=if(u1 ~= 0)
  Out1 : Outport  VectorParamsAs1DForOutWhenUnconnected=off
  wires:
  In1/1 -> Out1/1

== system CLVF/Phase #3: Experiment/Change BLACK Behavior/Sub-Phase #4/Lyapunov GNC/Navigation/x_dot -> x3/Hold this value ==
  In1 : Inport
  Action Port : ActionPort  ActionPortLabel=if(u1 ~= 0)
  Out1 : Outport  VectorParamsAs1DForOutWhenUnconnected=off
  wires:
  In1/1 -> Out1/1

== system CLVF/Phase #3: Experiment/Change BLACK Behavior/Sub-Phase #4/Lyapunov GNC/CLVF Approach/Vec Derivative/x_dot -> x1/Hold this value ==
  In1 : Inport
  Action Port : ActionPort  ActionPortLabel=if(u1 ~= 0)
  Out1 : Outport  VectorParamsAs1DForOutWhenUnconnected=off
  wires:
  In1/1 -> Out1/1

== system CLVF/Phase #3: Experiment/Change BLACK Behavior/Sub-Phase #4/Lyapunov GNC/CLVF Approach/Vec Derivative/x_dot -> x2/Hold this value ==
  In1 : Inport
  Action Port : ActionPort  ActionPortLabel=if(u1 ~= 0)
  Out1 : Outport  VectorParamsAs1DForOutWhenUnconnected=off
  wires:
  In1/1 -> Out1/1

== system CLVF/Phase #3: Experiment/Change BLACK Behavior/Sub-Phase #4/Lyapunov GNC/CLVF Approach/Vec Derivative/x_dot -> x3/Hold this value ==
  In1 : Inport
  Action Port : ActionPort  ActionPortLabel=if(u1 ~= 0)
  Out1 : Outport  VectorParamsAs1DForOutWhenUnconnected=off
  wires:
  In1/1 -> Out1/1

== system CLVF/Phase #3: Experiment/Change BLACK Behavior/Sub-Phase #4/Lyapunov GNC/Lyapunov/Vec Derivative/x_dot -> x1/Hold this value ==
  In1 : Inport
  Action Port : ActionPort  ActionPortLabel=if(u1 ~= 0)
  Out1 : Outport  VectorParamsAs1DForOutWhenUnconnected=off
  wires:
  In1/1 -> Out1/1

== system CLVF/Phase #3: Experiment/Change BLACK Behavior/Sub-Phase #4/Lyapunov GNC/Lyapunov/Vec Derivative/x_dot -> x2/Hold this value ==
  In1 : Inport
  Action Port : ActionPort  ActionPortLabel=if(u1 ~= 0)
  Out1 : Outport  VectorParamsAs1DForOutWhenUnconnected=off
  wires:
  In1/1 -> Out1/1

== system CLVF/Phase #3: Experiment/Change BLACK Behavior/Sub-Phase #4/Lyapunov GNC/Lyapunov/Vec Derivative/x_dot -> x3/Hold this value ==
  In1 : Inport
  Action Port : ActionPort  ActionPortLabel=if(u1 ~= 0)
  Out1 : Outport  VectorParamsAs1DForOutWhenUnconnected=off
  wires:
  In1/1 -> Out1/1

== system CLVF/Phase #3: Experiment/Change BLACK Behavior/Sub-Phase #4/Lyapunov GNC/Navigation/Vec Derivative/x_dot -> x1/Hold this value ==
  In1 : Inport
  Action Port : ActionPort  ActionPortLabel=if(u1 ~= 0)
  Out1 : Outport  VectorParamsAs1DForOutWhenUnconnected=off
  wires:
  In1/1 -> Out1/1

== system CLVF/Phase #3: Experiment/Change BLACK Behavior/Sub-Phase #4/Lyapunov GNC/Navigation/Vec Derivative/x_dot -> x2/Hold this value ==
  In1 : Inport
  Action Port : ActionPort  ActionPortLabel=if(u1 ~= 0)
  Out1 : Outport  VectorParamsAs1DForOutWhenUnconnected=off
  wires:
  In1/1 -> Out1/1

== system CLVF/Phase #3: Experiment/Change BLACK Behavior/Sub-Phase #4/Lyapunov GNC/Navigation/Vec Derivative/x_dot -> x3/Hold this value ==
  In1 : Inport
  Action Port : ActionPort  ActionPortLabel=if(u1 ~= 0)
  Out1 : Outport  VectorParamsAs1DForOutWhenUnconnected=off
  wires:
  In1/1 -> Out1/1

== system CLVF/Phase #3: Experiment/Change BLACK Behavior/Sub-Phase #4/Lyapunov GNC/Navigation/Vec Derivative1/x_dot -> x1/Hold this value ==
  In1 : Inport
  Action Port : ActionPort  ActionPortLabel=if(u1 ~= 0)
  Out1 : Outport  VectorParamsAs1DForOutWhenUnconnected=off
  wires:
  In1/1 -> Out1/1

== system CLVF/Phase #3: Experiment/Change BLACK Behavior/Sub-Phase #4/Lyapunov GNC/Navigation/Vec Derivative1/x_dot -> x2/Hold this value ==
  In1 : Inport
  Action Port : ActionPort  ActionPortLabel=if(u1 ~= 0)
  Out1 : Outport  VectorParamsAs1DForOutWhenUnconnected=off
  wires:
  In1/1 -> Out1/1

== system CLVF/Phase #3: Experiment/Change BLACK Behavior/Sub-Phase #4/Lyapunov GNC/Navigation/Vec Derivative1/x_dot -> x3/Hold this value ==
  In1 : Inport
  Action Port : ActionPort  ActionPortLabel=if(u1 ~= 0)
  Out1 : Outport  VectorParamsAs1DForOutWhenUnconnected=off
  wires:
  In1/1 -> Out1/1

== matlab function CLVF/Phase #2: Move to Initial Position/Change BLACK Behavior/Hough Control/MATLAB Function2 ==
  data: Oy output; z input; Ox output
function [Oy, Ox]   = C3( z )
%C3 gives the rotation matrix about the z-axis for an angle 'z'
%   z - the angle about the z-axis which you rotate
%   A - the rotation matrix

Ox = [cos(z) sin(z); -sin(z) cos(z)]*[1;0];
Oy = [cos(z) sin(z); -sin(z) cos(z)]*[0;1];
end

== matlab function CLVF/Phase #2: Move to Initial Position/Change BLACK Behavior/Hough Control/MATLAB Function3 ==
  data: z input; Ox output
function Ox    = C3( z )
%C3 gives the rotation matrix about the z-axis for an angle 'z'
%   z - the angle about the z-axis which you rotate
%   A - the rotation matrix

Ox = [cos(z) sin(z); -sin(z) cos(z)]*[1;0];
end

== matlab function CLVF/Phase #2: Move to Initial Position/Change BLACK Behavior/Hough Control/MATLAB Function4 ==
  data: Oy input; e_out output; e_in input
function e_out = fcn(Oy, e_in)

a = sign(Oy'*e_in);
e_out = -a*norm(e_in);

== matlab function CLVF/From Force//Torque to PWM Signal/Change BLACK Behavior/Calculate Thruster ON//OFF/MATLAB Function ==
  data: H output; thruster_dist2CG_BLACK parameter; F_thrusters_BLACK parameter
function H = MakeH(thruster_dist2CG_BLACK,F_thrusters_BLACK)

Vec1 = [ -1
         -1
          0 
          0
          1
          1
          0
          0 ];
      
Vec2 = [  0
          0
          1
          1
          0
          0
         -1
         -1 ];
     
Vec3 = thruster_dist2CG_BLACK./1000;

Mat1 = [Vec1, Vec2, Vec3]';

Mat2 = diag((F_thrusters_BLACK./2));

H    = Mat1*Mat2;

end

== matlab function CLVF/Phase #3: Experiment/Change BLACK Behavior/Sub-Phase #4/BLACK_RzD/Wrap1/MATLAB Function ==
  data: u input; wrappedAngle output
function wrappedAngle = wrapAngle(u)

wrappedAngle = atan2(sin(u),cos(u));

end

== matlab function CLVF/Phase #3: Experiment/Change BLACK Behavior/Sub-Phase #4/Hough Control/MATLAB Function2 ==
  data: Oy output; z input; Ox output
function [Oy, Ox]   = C3( z )
%C3 gives the rotation matrix about the z-axis for an angle 'z'
%   z - the angle about the z-axis which you rotate
%   A - the rotation matrix

Ox = [cos(z) sin(z); -sin(z) cos(z)]*[1;0];
Oy = [cos(z) sin(z); -sin(z) cos(z)]*[0;1];
end

== matlab function CLVF/From Force//Torque to PWM Signal/Change BLACK Behavior/Calculate Thruster ON//OFF/MATLAB Function1 ==
  data: H output; thruster_dist2CG_BLACK parameter; F_thrusters_BLACK parameter
function H = MakeH(thruster_dist2CG_BLACK,F_thrusters_BLACK)

Vec1 = [ -1
         -1
          0 
          0
          1
          1
          0
          0 ];
      
Vec2 = [  0
          0
          1
          1
          0
          0
         -1
         -1 ];
     
Vec3 = thruster_dist2CG_BLACK./1000;

Mat1 = [Vec1, Vec2, Vec3]';

Mat2 = diag((F_thrusters_BLACK));

H    = Mat1*Mat2;

end

== matlab function CLVF/From Force//Torque to PWM Signal/Change BLACK Behavior/Calculate Thruster ON//OFF/MATLAB Function2 ==
  data: ThrustPer_Final output; ThrustPer input
function ThrustPer_Final  = ThrusterSat(ThrustPer)

ValveTime       = 0.007;
TControl        = 0.1;
ThrustPer_Final = zeros(8,1);

if max(ThrustPer) > 1
    ThrustPer_Sat = ThrustPer/max(ThrustPer);
else
    ThrustPer_Sat = ThrustPer;
end

for i = 1:8
    if ThrustPer_Sat(i) > ValveTime/TControl 
        ThrustPer_Final(i) = ThrustPer_Sat(i);
    else
        ThrustPer_Final(i) = 0;
    end
end
   

end

== matlab function CLVF/From Force//Torque to PWM Signal/Change BLACK Behavior/Calculate Thruster ON//OFF/Rotate Forces to Inertial/Create Rotation Matrix ==
  data: Rz input; C_Ib output
function C_Ib = RotateFrame(Rz)

C_bI = [  cos(Rz) sin(Rz)
         -sin(Rz) cos(Rz) ];

C_Ib = inv(C_bI);

end

== matlab function CLVF/From Force//Torque to PWM Signal/Change BLACK Behavior/Rotate Forces to Body/Create Rotation Matrix ==
  data: Rz input; C_bI output
function C_bI = RotateFrame(Rz)

C_bI = [  cos(Rz) sin(Rz)
         -sin(Rz) cos(Rz) ];

end

== matlab function CLVF/From Force//Torque to PWM Signal/Change RED Behavior/Calculate Thruster ON//OFF/MATLAB Function ==
  data: H output; thruster_dist2CG_RED parameter; F_thrusters_RED parameter
function H = MakeH(thruster_dist2CG_RED,F_thrusters_RED)

Vec1 = [ -1
         -1
          0 
          0
          1
          1
          0
          0 ];
      
Vec2 = [  0
          0
          1
          1
          0
          0
         -1
         -1 ];
     
Vec3 = thruster_dist2CG_RED./1000;

Mat1 = [Vec1, Vec2, Vec3]';

Mat2 = diag((F_thrusters_RED./2));

H    = Mat1*Mat2;

end

== matlab function CLVF/From Force//Torque to PWM Signal/Change RED Behavior/Calculate Thruster ON//OFF/MATLAB Function1 ==
  data: H output; thruster_dist2CG_RED parameter; F_thrusters_RED parameter
function H = MakeH(thruster_dist2CG_RED,F_thrusters_RED)

Vec1 = [ -1
         -1
          0 
          0
          1
          1
          0
          0 ];
      
Vec2 = [  0
          0
          1
          1
          0
          0
         -1
         -1 ];
     
Vec3 = thruster_dist2CG_RED./1000;

Mat1 = [Vec1, Vec2, Vec3]';

Mat2 = diag((F_thrusters_RED));

H    = Mat1*Mat2;

end

== matlab function CLVF/From Force//Torque to PWM Signal/Change RED Behavior/Calculate Thruster ON//OFF/MATLAB Function2 ==
  data: ThrustPer_Final output; ThrustPer input
function ThrustPer_Final  = ThrusterSat(ThrustPer)

ValveTime       = 0.007;
TControl        = 0.1;
ThrustPer_Final = zeros(8,1);

if max(ThrustPer) > 1
    ThrustPer_Sat = ThrustPer/max(ThrustPer);
else
    ThrustPer_Sat = ThrustPer;
end

for i = 1:8
    if ThrustPer_Sat(i) > ValveTime/TControl 
        ThrustPer_Final(i) = ThrustPer_Sat(i);
    else
        ThrustPer_Final(i) = 0;
    end
end
   

end

== matlab function CLVF/From Force//Torque to PWM Signal/Change RED Behavior/Calculate Thruster ON//OFF/Rotate Forces to Inertial/Create Rotation Matrix ==
  data: Rz input; C_Ib output
function C_Ib = RotateFrame(Rz)

C_bI = [  cos(Rz) sin(Rz)
         -sin(Rz) cos(Rz) ];

C_Ib = inv(C_bI);

end

== matlab function CLVF/Simulate Plant Dynamics/Sample and Hold Data to Match PhaseSpace (RED)/MATLAB Function ==
  data: TIME input; y output; SERVER input
function y = fcn(TIME, SERVER)

if mod(TIME,SERVER) == 0
    y = 1;
else
    y = 0;
end

== matlab function CLVF/Simulate Plant Dynamics/Sample and Hold Data to Match PhaseSpace (BLACK)/MATLAB Function ==
  data: TIME input; y output; SERVER input
function y = fcn(TIME, SERVER)

if mod(TIME,SERVER) == 0
    y = 1;
else
    y = 0;
end

== matlab function CLVF/From Force//Torque to PWM Signal/Change RED Behavior/Rotate Forces to Body/Create Rotation Matrix ==
  data: Rz input; C_bI output
function C_bI = RotateFrame(Rz)

C_bI = [  cos(Rz) sin(Rz)
         -sin(Rz) cos(Rz) ];

end

== matlab function CLVF/Phase #2: Move to Initial Position/Change RED Behavior/Hough Control/MATLAB Function2 ==
  data: Oy output; z input; Ox output
function [Oy, Ox]   = C3( z )
%C3 gives the rotation matrix about the z-axis for an angle 'z'
%   z - the angle about the z-axis which you rotate
%   A - the rotation matrix

Ox = [cos(z) sin(z); -sin(z) cos(z)]*[1;0];
Oy = [cos(z) sin(z); -sin(z) cos(z)]*[0;1];
end

== matlab function CLVF/Phase #2: Move to Initial Position/Change RED Behavior/Hough Control/MATLAB Function3 ==
  data: z input; Ox output
function Ox    = C3( z )
%C3 gives the rotation matrix about the z-axis for an angle 'z'
%   z - the angle about the z-axis which you rotate
%   A - the rotation matrix

Ox = [cos(z) sin(z); -sin(z) cos(z)]*[1;0];
end

== matlab function CLVF/Phase #2: Move to Initial Position/Change RED Behavior/Hough Control/MATLAB Function4 ==
  data: Oy input; e_out output; e_in input
function e_out = fcn(Oy, e_in)

a = sign(Oy'*e_in);
e_out = -a*norm(e_in);

== matlab function CLVF/Phase #3: Experiment/Change BLACK Behavior/Sub-Phase #4/Hough Control/MATLAB Function3 ==
  data: z input; Ox output
function Ox    = C3( z )
%C3 gives the rotation matrix about the z-axis for an angle 'z'
%   z - the angle about the z-axis which you rotate
%   A - the rotation matrix

Ox = [cos(z) sin(z); -sin(z) cos(z)]*[1;0];
end

== matlab function CLVF/Phase #4: Return Home/Change BLACK Behavior/Hough Control/MATLAB Function2 ==
  data: Oy output; z input; Ox output
function [Oy, Ox]   = C3( z )
%C3 gives the rotation matrix about the z-axis for an angle 'z'
%   z - the angle about the z-axis which you rotate
%   A - the rotation matrix

Ox = [cos(z) sin(z); -sin(z) cos(z)]*[1;0];
Oy = [cos(z) sin(z); -sin(z) cos(z)]*[0;1];
end

== matlab function CLVF/Phase #4: Return Home/Change BLACK Behavior/Hough Control/MATLAB Function3 ==
  data: z input; Ox output
function Ox    = C3( z )
%C3 gives the rotation matrix about the z-axis for an angle 'z'
%   z - the angle about the z-axis which you rotate
%   A - the rotation matrix

Ox = [cos(z) sin(z); -sin(z) cos(z)]*[1;0];
end

== matlab function CLVF/Phase #4: Return Home/Change BLACK Behavior/Hough Control/MATLAB Function4 ==
  data: Oy input; e_out output; e_in input
function e_out = fcn(Oy, e_in)

a = sign(Oy'*e_in);
e_out = -a*norm(e_in);

== matlab function CLVF/Phase #4: Return Home/Change RED Behavior/Hough Control/MATLAB Function2 ==
  data: Oy output; z input; Ox output
function [Oy, Ox]   = C3( z )
%C3 gives the rotation matrix about the z-axis for an angle 'z'
%   z - the angle about the z-axis which you rotate
%   A - the rotation matrix

Ox = [cos(z) sin(z); -sin(z) cos(z)]*[1;0];
Oy = [cos(z) sin(z); -sin(z) cos(z)]*[0;1];
end

== matlab function CLVF/Phase #4: Return Home/Change RED Behavior/Hough Control/MATLAB Function3 ==
  data: z input; Ox output
function Ox    = C3( z )
%C3 gives the rotation matrix about the z-axis for an angle 'z'
%   z - the angle about the z-axis which you rotate
%   A - the rotation matrix

Ox = [cos(z) sin(z); -sin(z) cos(z)]*[1;0];
end

== matlab function CLVF/Phase #4: Return Home/Change RED Behavior/Hough Control/MATLAB Function4 ==
  data: Oy input; e_out output; e_in input
function e_out = fcn(Oy, e_in)

a = sign(Oy'*e_in);
e_out = -a*norm(e_in);

== matlab function CLVF/Phase #2: Move to Initial Position/Change BLUE Behavior/Hough Control/MATLAB Function2 ==
  data: Oy output; z input; Ox output
function [Oy, Ox]   = C3( z )
%C3 gives the rotation matrix about the z-axis for an angle 'z'
%   z - the angle about the z-axis which you rotate
%   A - the rotation matrix

Ox = [cos(z) sin(z); -sin(z) cos(z)]*[1;0];
Oy = [cos(z) sin(z); -sin(z) cos(z)]*[0;1];
end

== matlab function CLVF/Phase #2: Move to Initial Position/Change BLUE Behavior/Hough Control/MATLAB Function3 ==
  data: z input; Ox output
function Ox    = C3( z )
%C3 gives the rotation matrix about the z-axis for an angle 'z'
%   z - the angle about the z-axis which you rotate
%   A - the rotation matrix

Ox = [cos(z) sin(z); -sin(z) cos(z)]*[1;0];
end
